simulink model "dcdc1"  (R2024a)
settings: Solver=ode15s  StartTime=0.0  StopTime=0.2  MaxStep=1/20e6  RelTol=1e-3  EnableMultiTasking=on
undefined symbols (not defined in the file): C, C0, L, L0, R, Vin
libraries: spsGroundLib x5, simulink_need_slupdate x2, spsSeriesRLCBranchLib x2, spsVoltageMeasurementLib x2, spsCurrentMeasurementLib x1, spsDCVoltageSourceLib x1, spsDiodeLib x1, spsIdealSwitchLib x1, spsMeanLib x1, spsPWMGeneratorDCDCLib x1, spsParallelRLCBranchLib x1, sps_lib x1
settings Model: Creator=almazaya  LastModifiedBy=ashra
settings SolverCC: ZeroCrossAlgorithm=Non-adaptive  AlgebraicLoopSolver=TrustRegion
settings DataIOCC: LimitDataPoints=on  SaveFormat=Array  SignalLoggingSaveFormat=ModelDataLogs  ReturnWorkspaceOutputs=off
settings OptimizationCC: ExpressionDepthLimit=2147483647  InitFltsAndDblsToZero=on  LifeSpan=inf
settings DebuggingCC: UnderspecifiedInitializationDetection=Classic  MergeDetectMultiDrivingBlocksExec=none  SolverPrmCheckMsg=warning  FcnCallInpInsideContextMsg=warning  UnconnectedInputMsg=warning  UnconnectedOutputMsg=warning  UnconnectedLineMsg=warning  StateNameClashWarn=warning  SFUnexpectedBacktrackingDiag=warning  SFNoUnconditionalDefaultTransitionDiag=warning  SFExecutionAtInitializationDiag=none  ArithmeticOperatorsInVariantConditions=warning
settings HardwareCC: ProdBitPerPointer=32  ProdBitPerSizeT=32  ProdBitPerPtrDiffT=32  ProdLargestAtomicFloat=None  ProdIntDivRoundTo=Undefined  ProdEndianess=Unspecified  ProdWordSize=32  ProdHWDeviceType=32-bit Generic
settings ModelReferenceCC: PropagateSignalLabelsOutOfModel=off
settings RTWCC: GPUComputeCapability=3.5
settings CodeAppCC: StateflowObjectComments=on
settings GRTTargetCC: TargetLangStandard=C89/C90 (ANSI)  CombineOutputUpdateFcns=off  GRTInterface=on
settings ConfigComp: CovMetricSettings=dw  CovSaveCumulativeToWorkspaceVar=on  CovSaveSingleToWorkspaceVar=on

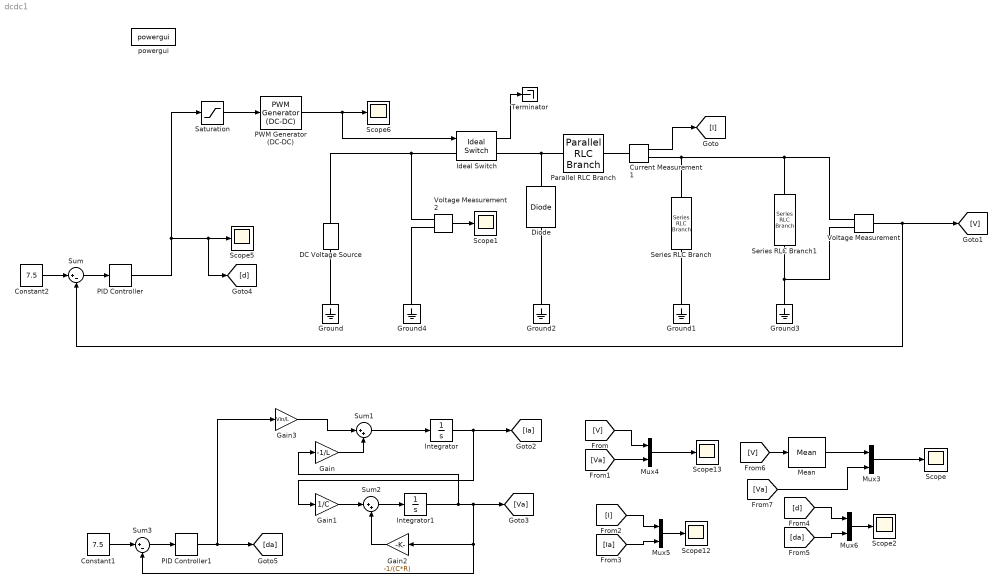
== system dcdc1 ==
  Constant1 : Constant  Value=7.5
  Constant2 : Constant  Value=7.5
  Current Measurement1 : spsCurrentMeasurementLib/Current Measurement  PhasorSimulation=off  OutputType=Complex  PSBequivalent=0
  DC Voltage Source : spsDCVoltageSourceLib/DC Voltage Source  Amplitude=Vin  Measurements=None
  Diode : spsDiodeLib/Diode  Ron=1e-6  Lon=0  Vf=0  IC=0  UseSnubber=off  Rs=inf  Cs=0  Measurements=off
  Gain : Gain  Gain=-1/L
  Gain1 : Gain  Gain=1/C
  Gain2 : Gain  Gain=-1/(C*R)
  Gain3 : Gain  Gain=Vin/L
  Ground{,1..4} (5 alike) : spsGroundLib/Ground  LConnTagsString=a
  Ideal Switch : spsIdealSwitchLib/Ideal Switch  Ron=0.001  Lon=0  IC=0  Rs=1e5  Cs=inf  Measurements=on
  Integrator : Integrator  InitialCondition=L0
  Integrator1 : Integrator  InitialCondition=C0
  Mean : spsMeanLib/Mean  Freq=f  Vinit=7  Ts=0
  Mux{3..6} (4 alike) : Mux  Inputs=2
  PID Controller : simulink_need_slupdate/PID Controller  P=1  I=10  D=0
  PID Controller1 : simulink_need_slupdate/PID Controller  P=1  I=10  D=0
  PWM Generator (DC-DC) : spsPWMGeneratorDCDCLib/PWM Generator (DC-DC)  Fsw=f  Ts=0
  Parallel RLC Branch : spsParallelRLCBranchLib/Parallel RLC Branch  LConnTagsString=a  RConnTagsString=__new0  BranchType=L  Resistance=1  Inductance=L  SetiL0=on  InitialCurrent=L0  Capacitance=1e-6  Setx0=off  InitialVoltage=0  Measurements=None
  Saturation : Saturate  UpperLimit=1  LowerLimit=0
  Scope{,1..2,5..6,12..13} (7 alike) : Scope
  Series RLC Branch : spsSeriesRLCBranchLib/Series RLC Branch  LConnTagsString=__new0  RConnTagsString=__new0  BranchType=C  Resistance=1  Inductance=1e-3  SetiL0=off  InitialCurrent=0  Capacitance=C  Setx0=on  InitialVoltage=C0  Measurements=None
  Series RLC Branch1 : spsSeriesRLCBranchLib/Series RLC Branch  LConnTagsString=__new0  RConnTagsString=__new0  BranchType=R  Resistance=R  Inductance=1e-3  SetiL0=off  InitialCurrent=0  Capacitance=1e-6  Setx0=off  InitialVoltage=0  Measurements=Branch voltage
  Sum : Sum  Inputs=|+-
  Sum1 : Sum  Inputs=|++
  Sum2 : Sum  Inputs=|++
  Sum3 : Sum  Inputs=|+-
  Terminator : Terminator
  Voltage Measurement : spsVoltageMeasurementLib/Voltage Measurement  PhasorSimulation=off  OutputType=Complex  PSBequivalent=0
  Voltage Measurement2 : spsVoltageMeasurementLib/Voltage Measurement  PhasorSimulation=off  OutputType=Complex  PSBequivalent=0
  powergui : sps_lib/powergui  SimulationMode=Continuous  SampleTime=1e-5  frequency=60  Iterations=50  frequencyindice=0  Pbase=100e6  ErrMax=1e-4  UnitsV=kV  UnitsW=MW  buscounter=0  FunctionMessages=off  echomessages=off  EnableUseOfTLC=off  CurrentSourceSwitches=off  DisableSnubberDevices=off  DisableRonSwitches=off  DisableVfSwitches=off  DisplayEquations=off  AutomaticDiscreteSolvers=off  SolverType=Tustin/Backward Euler (TBE)  Interpol=off  ExternalGateDelay=off  methode=off  Ts=0  x0status=blocks  SPID=off  SwTol=0  HookPort=off  NonlinearTolerance=1e-4  nMaxIteration=100  ContinueOnMaxIteration=off  RestoreLinks=warning  ResistiveCurrentMeasurement=off  Frange=[0:2:500]  Ylog=off  Xlog=on  ShowGrid=off  save=off  variable=ZData  structure=0  ZoomFFT=on  StartTime=0.0  cycles=1  DisplayStyle=1  fundamental=60  FreqAxis=off  MaxFrequency=1000  frequencyindicesteady=1  RmsSteady=1  display=off
  wires:
  Ideal Switch/1 -> Terminator/1
  Voltage Measurement/1 -> [V], Sum/2
  Voltage Measurement2/1 -> Scope1/1
  Constant2/1 -> Sum/1
  PID Controller/1 -> [d], Scope5/1, Saturation/1
  Sum/1 -> PID Controller/1
  Saturation/1 -> PWM Generator (DC-DC)/1
  PWM Generator (DC-DC)/1 -> Ideal Switch/1, Scope6/1
  Sum1/1 -> Integrator/1
  Gain/1 -> Sum1/2
  Integrator/1 -> [Ia], Gain1/1
  Gain1/1 -> Sum2/1
  Sum2/1 -> Integrator1/1
  Gain2/1 -> Sum2/2
  Constant1/1 -> Sum3/1
  Sum3/1 -> PID Controller1/1
  Gain3/1 -> Sum1/1
  PID Controller1/1 -> Gain3/1, [da]
  Integrator1/1 -> Gain/1, [Va], Gain2/1, Sum3/2
  Mean/1 -> Mux3/1
  Mux5/1 -> Scope12/1
  [V] -> Mux4/1
  [I] -> Mux5/1
  [Va] -> Mux4/2
  Mux4/1 -> Scope13/1
  [Ia] -> Mux5/2
  Current Measurement1/1 -> [I]
  Mux3/1 -> Scope/1
  [da] -> Mux6/2
  [d] -> Mux6/1
  Mux6/1 -> Scope2/1
  [V] -> Mean/1
  [Va] -> Mux3/2
  connections:
  Voltage Measurement/LConn2 -- Ground3/LConn1 -- Series RLC Branch1/RConn1
  Current Measurement1/RConn1 -- Voltage Measurement/LConn1 -- Series RLC Branch1/LConn1 -- Series RLC Branch/LConn1
  Diode/RConn1 -- Parallel RLC Branch/LConn1 -- Ideal Switch/RConn1
  Ground/LConn1 -- DC Voltage Source/LConn1
  Ideal Switch/LConn1 -- DC Voltage Source/RConn1 -- Voltage Measurement2/LConn1
  Ground4/LConn1 -- Voltage Measurement2/LConn2
  Parallel RLC Branch/RConn1 -- Current Measurement1/LConn1
  Ground2/LConn1 -- Diode/LConn1
  Series RLC Branch/RConn1 -- Ground1/LConn1
